simulink model "SoftGripperPick"  (R2026b)
settings: Solver=daessc  StopTime=16  RelTol=1e-4
undefined symbols (not defined in the file): magnitude, P, X, Y, Z
libraries: sm_lib x123, nesl_utility x40, fl_lib x4
(part 3 of 3)

== system SoftGripperPick/Plant/UR5e/wrist_2_link ==
  Inertia : sm_lib/Body Elements/Inertia  InertiaType=Custom  Mass=1.3  MassUnits=kg  CenterOfMass=[0, 0, 0]  CenterOfMassUnits=m  MomentsOfInertia=[0.00135617, 0.00096614, 0.00127827]  MomentsOfInertiaUnits=kg*m^2  ProductsOfInertia=[5.048000000000011e-05, 2.739999999999998e-06, 4.440000000000001e-06]  ProductsOfInertiaUnits=kg*m^2  GraphicType=None  MarkerShape=Inertia  MarkerSize=20  GraphicVisPropType=SimpleVisualProperties  GraphicDiffuseColor=[0.5 0.5 0.5]  GraphicOpacity=1  GraphicSpecularColor=[0.5 0.5 0.5 1.0]  GraphicAmbientColor=[0.15 0.15 0.15 1.0]  GraphicEmissiveColor=[0.0 0.0 0.0 1.0]  GraphicShininess=75
  InertiaOriginTransform : sm_lib/Frames and Transforms/Rigid Transform  RotationMethod=RotationSequence  FollAlignAxisA=+X  BaseAlignAxisA=+Y  FollAlignAxisB=+Y  BaseAlignAxisB=+Z  RotationStandardAxis=+Z  RotationAngle=0  RotationAngleUnits=deg  RotationArbitraryAxis=[0 0 1]  RotationSequenceAxes=BaseAxes  RotationSequence=XYZ  RotationSequenceAngles=[0, 0, 0]  RotationSequenceAnglesUnits=rad  RotationMatrix=[1 0 0;0 1 0;0 0 1]  Quaternion=[1 0 0 0]  TranslationMethod=Cartesian  TranslationCartesianOffset=[0, 0.01634, -0.0018]  TranslationCartesianOffsetUnits=m  TranslationStandardAxis=+Z  TranslationStandardOffset=0  TranslationStandardOffsetUnits=m  TranslationROffset=0  TranslationROffsetUnits=m  TranslationThetaOffset=0  TranslationThetaOffsetUnits=deg  TranslationZOffset=0  TranslationZOffsetUnits=m
  ReferenceFrame : sm_lib/Frames and Transforms/Reference Frame
  wrist_2_joint_AxisInvTransform : sm_lib/Frames and Transforms/Rigid Transform  RotationMethod=ArbitraryAxis  FollAlignAxisA=+X  BaseAlignAxisA=+Y  FollAlignAxisB=+Y  BaseAlignAxisB=+Z  RotationStandardAxis=+Z  RotationAngle=0  RotationAngleUnits=rad  RotationArbitraryAxis=[1, 0, 0]  RotationSequenceAxes=FollowerAxes  RotationSequence=XYX  RotationSequenceAngles=[0 0 0]  RotationSequenceAnglesUnits=deg  RotationMatrix=[1 0 0;0 1 0;0 0 1]  Quaternion=[1 0 0 0]  TranslationMethod=Cartesian  TranslationCartesianOffset=[0, 0, 0]  TranslationCartesianOffsetUnits=m  TranslationStandardAxis=+Z  TranslationStandardOffset=0  TranslationStandardOffsetUnits=m  TranslationROffset=0  TranslationROffsetUnits=m  TranslationThetaOffset=0  TranslationThetaOffsetUnits=deg  TranslationZOffset=0  TranslationZOffsetUnits=m
  wrist_3_joint_AxisTransform : sm_lib/Frames and Transforms/Rigid Transform  RotationMethod=ArbitraryAxis  FollAlignAxisA=+X  BaseAlignAxisA=+Y  FollAlignAxisB=+Y  BaseAlignAxisB=+Z  RotationStandardAxis=+Z  RotationAngle=0  RotationAngleUnits=rad  RotationArbitraryAxis=[1, 0, 0]  RotationSequenceAxes=FollowerAxes  RotationSequence=XYX  RotationSequenceAngles=[0 0 0]  RotationSequenceAnglesUnits=deg  RotationMatrix=[1 0 0;0 1 0;0 0 1]  Quaternion=[1 0 0 0]  TranslationMethod=Cartesian  TranslationCartesianOffset=[0, 0, 0]  TranslationCartesianOffsetUnits=m  TranslationStandardAxis=+Z  TranslationStandardOffset=0  TranslationStandardOffsetUnits=m  TranslationROffset=0  TranslationROffsetUnits=m  TranslationThetaOffset=0  TranslationThetaOffsetUnits=deg  TranslationZOffset=0  TranslationZOffsetUnits=m
  wrist_3_joint_OriginTransform : sm_lib/Frames and Transforms/Rigid Transform  RotationMethod=RotationSequence  FollAlignAxisA=+X  BaseAlignAxisA=+Y  FollAlignAxisB=+Y  BaseAlignAxisB=+Z  RotationStandardAxis=+Z  RotationAngle=0  RotationAngleUnits=deg  RotationArbitraryAxis=[0 0 1]  RotationSequenceAxes=BaseAxes  RotationSequence=XYZ  RotationSequenceAngles=[-1.570796327, 1.224646799147353e-16, -1.224646799147353e-16]  RotationSequenceAnglesUnits=rad  RotationMatrix=[1 0 0;0 1 0;0 0 1]  Quaternion=[1 0 0 0]  TranslationMethod=Cartesian  TranslationCartesianOffset=[0, 0.09959999999999999, -2.042830148012698e-11]  TranslationCartesianOffsetUnits=m  TranslationStandardAxis=+Z  TranslationStandardOffset=0  TranslationStandardOffsetUnits=m  TranslationROffset=0  TranslationROffsetUnits=m  TranslationThetaOffset=0  TranslationThetaOffsetUnits=deg  TranslationZOffset=0  TranslationZOffsetUnits=m
  F : PMIOPort  Side=Left
  F1 : PMIOPort  Port=2  Side=Right
  connections:
  wrist_3_joint_AxisTransform/LConn1 -- wrist_3_joint_OriginTransform/RConn1
  wrist_3_joint_AxisTransform/RConn1 -- F1/RConn1
  wrist_2_joint_AxisInvTransform/RConn1 -- F/RConn1
  wrist_3_joint_OriginTransform/LConn1 -- wrist_2_joint_AxisInvTransform/LConn1 -- ReferenceFrame/RConn1 -- InertiaOriginTransform/LConn1
  Inertia/RConn1 -- InertiaOriginTransform/RConn1

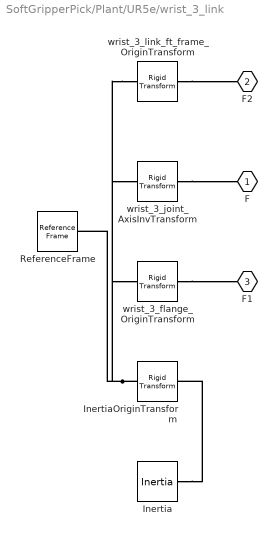
== system SoftGripperPick/Plant/UR5e/wrist_3_link ==
  Inertia : sm_lib/Body Elements/Inertia  InertiaType=Custom  Mass=0.365  MassUnits=kg  CenterOfMass=[0, 0, 0]  CenterOfMassUnits=m  MomentsOfInertia=[0.00018694, 0.00018908, 0.00025756]  MomentsOfInertiaUnits=kg*m^2  ProductsOfInertia=[-9.2e-07, -1.7e-07, 5.999999999999999e-08]  ProductsOfInertiaUnits=kg*m^2  GraphicType=None  MarkerShape=Inertia  MarkerSize=20  GraphicVisPropType=SimpleVisualProperties  GraphicDiffuseColor=[0.5 0.5 0.5]  GraphicOpacity=1  GraphicSpecularColor=[0.5 0.5 0.5 1.0]  GraphicAmbientColor=[0.15 0.15 0.15 1.0]  GraphicEmissiveColor=[0.0 0.0 0.0 1.0]  GraphicShininess=75
  InertiaOriginTransform : sm_lib/Frames and Transforms/Rigid Transform  RotationMethod=RotationSequence  FollAlignAxisA=+X  BaseAlignAxisA=+Y  FollAlignAxisB=+Y  BaseAlignAxisB=+Z  RotationStandardAxis=+Z  RotationAngle=0  RotationAngleUnits=deg  RotationArbitraryAxis=[0 0 1]  RotationSequenceAxes=BaseAxes  RotationSequence=XYZ  RotationSequenceAngles=[0, 0, 0]  RotationSequenceAnglesUnits=rad  RotationMatrix=[1 0 0;0 1 0;0 0 1]  Quaternion=[1 0 0 0]  TranslationMethod=Cartesian  TranslationCartesianOffset=[0, 0, -0.001159]  TranslationCartesianOffsetUnits=m  TranslationStandardAxis=+Z  TranslationStandardOffset=0  TranslationStandardOffsetUnits=m  TranslationROffset=0  TranslationROffsetUnits=m  TranslationThetaOffset=0  TranslationThetaOffsetUnits=deg  TranslationZOffset=0  TranslationZOffsetUnits=m
  ReferenceFrame : sm_lib/Frames and Transforms/Reference Frame
  wrist_3_flange_OriginTransform : sm_lib/Frames and Transforms/Rigid Transform  RotationMethod=RotationSequence  FollAlignAxisA=+X  BaseAlignAxisA=+Y  FollAlignAxisB=+Y  BaseAlignAxisB=+Z  RotationStandardAxis=+Z  RotationAngle=0  RotationAngleUnits=deg  RotationArbitraryAxis=[0 0 1]  RotationSequenceAxes=BaseAxes  RotationSequence=XYZ  RotationSequenceAngles=[-1.570796326794897, -1.570796326794897, 0]  RotationSequenceAnglesUnits=rad  RotationMatrix=[1 0 0;0 1 0;0 0 1]  Quaternion=[1 0 0 0]  TranslationMethod=Cartesian  TranslationCartesianOffset=[0, 0, 0]  TranslationCartesianOffsetUnits=m  TranslationStandardAxis=+Z  TranslationStandardOffset=0  TranslationStandardOffsetUnits=m  TranslationROffset=0  TranslationROffsetUnits=m  TranslationThetaOffset=0  TranslationThetaOffsetUnits=deg  TranslationZOffset=0  TranslationZOffsetUnits=m
  wrist_3_joint_AxisInvTransform : sm_lib/Frames and Transforms/Rigid Transform  RotationMethod=ArbitraryAxis  FollAlignAxisA=+X  BaseAlignAxisA=+Y  FollAlignAxisB=+Y  BaseAlignAxisB=+Z  RotationStandardAxis=+Z  RotationAngle=0  RotationAngleUnits=rad  RotationArbitraryAxis=[1, 0, 0]  RotationSequenceAxes=FollowerAxes  RotationSequence=XYX  RotationSequenceAngles=[0 0 0]  RotationSequenceAnglesUnits=deg  RotationMatrix=[1 0 0;0 1 0;0 0 1]  Quaternion=[1 0 0 0]  TranslationMethod=Cartesian  TranslationCartesianOffset=[0, 0, 0]  TranslationCartesianOffsetUnits=m  TranslationStandardAxis=+Z  TranslationStandardOffset=0  TranslationStandardOffsetUnits=m  TranslationROffset=0  TranslationROffsetUnits=m  TranslationThetaOffset=0  TranslationThetaOffsetUnits=deg  TranslationZOffset=0  TranslationZOffsetUnits=m
  wrist_3_link_ft_frame_OriginTransform : sm_lib/Frames and Transforms/Rigid Transform  RotationMethod=RotationSequence  FollAlignAxisA=+X  BaseAlignAxisA=+Y  FollAlignAxisB=+Y  BaseAlignAxisB=+Z  RotationStandardAxis=+Z  RotationAngle=0  RotationAngleUnits=deg  RotationArbitraryAxis=[0 0 1]  RotationSequenceAxes=BaseAxes  RotationSequence=XYZ  RotationSequenceAngles=[3.141592653589793, -0, 0]  RotationSequenceAnglesUnits=rad  RotationMatrix=[1 0 0;0 1 0;0 0 1]  Quaternion=[1 0 0 0]  TranslationMethod=Cartesian  TranslationCartesianOffset=[0, 0, 0]  TranslationCartesianOffsetUnits=m  TranslationStandardAxis=+Z  TranslationStandardOffset=0  TranslationStandardOffsetUnits=m  TranslationROffset=0  TranslationROffsetUnits=m  TranslationThetaOffset=0  TranslationThetaOffsetUnits=deg  TranslationZOffset=0  TranslationZOffsetUnits=m
  F : PMIOPort  Side=Left
  F2 : PMIOPort  Port=2  Side=Right
  F1 : PMIOPort  Port=3  Side=Right
  connections:
  wrist_3_link_ft_frame_OriginTransform/RConn1 -- F2/RConn1
  wrist_3_joint_AxisInvTransform/RConn1 -- F/RConn1
  wrist_3_flange_OriginTransform/RConn1 -- F1/RConn1
  wrist_3_link_ft_frame_OriginTransform/LConn1 -- wrist_3_joint_AxisInvTransform/LConn1 -- wrist_3_flange_OriginTransform/LConn1 -- ReferenceFrame/RConn1 -- InertiaOriginTransform/LConn1
  Inertia/RConn1 -- InertiaOriginTransform/RConn1

== stateflow chart SoftGripperPick/Controller/PickTask ==
  settings: updateMethod=DISCRETE  sampleTime=P.ctrl.Ts_Ctrl
  state Active
    en: Ts = taskCfg(1); pGrip = gripCfg(1); tMax = taskCfg(5);
    tTot = 0; attempt = 1; supplyLow = 0; lowCnt = 0; pCmd = 0; qCmd = qHome;
    du: tTot = tTot + Ts;
    if pCmd >= pGrip && pMeas < pGrip - gripCfg(6), lowCnt = lowCnt + 1; else, lowCnt = 0; end
    if lowCnt * Ts >= gripCfg(7), supplyLow = 1; end
    state Settle
      en: qCmd = qHome; pCmd = 0;
    state Approach
      en: tSeg = 0;
      du: tSeg = tSeg + Ts; qCmd = traj(segQ0(1,:), segQ1(1,:), segT(1), tSeg);
    state Descend
      en: tSeg = 0;
      du: tSeg = tSeg + Ts; qCmd = traj(segQ0(2,:), segQ1(2,:), segT(2), tSeg);
    state Close
      en: tC = 0; stallCnt = 0; stalled = 0; bendPrev = bend;
      du: tC = tC + Ts; pCmd = min(pGrip, pGrip * tC / gripCfg(3)); stallCnt = stallCnt + 1;
      if stallCnt >= detCfg(3), stalled = double(all(abs(bend - bendPrev) / (stallCnt * Ts) < detCfg(2))); bendPrev = bend; stallCnt = 0; end
    state CheckGrasp
      en: nContact = countContact(bend, pMeas, bendTab, detCfg);
    state Lift
      en: tSeg = 0;
      du: tSeg = tSeg + Ts; qCmd = traj(segQ0(3,:), segQ1(3,:), segT(3), tSeg);
    state Transport
      en: tSeg = 0;
      du: tSeg = tSeg + Ts; qCmd = traj(segQ0(4,:), segQ1(4,:), segT(4), tSeg);
    state Lower
      en: tSeg = 0;
      du: tSeg = tSeg + Ts; qCmd = traj(segQ0(5,:), segQ1(5,:), segT(5), tSeg);
    state Retry
      en: attempt = attempt + 1; pCmd = 0; tSeg = 0; qStart = qMeas;
      du: tSeg = tSeg + Ts; qCmd = traj(qStart, segQ0(2,:), max(segT), tSeg);
    state Release
      en: pCmd = 0;
    state Retreat
      en: tSeg = 0;
      du: tSeg = tSeg + Ts; qCmd = traj(segQ0(6,:), segQ1(6,:), segT(6), tSeg);
    (default) -> Settle
    Settle -> Approach : [after(taskCfg(2), sec)]
    Approach -> Descend : [tSeg >= segT(1) && arrived(qMeas, segQ1(1,:), taskCfg(3))]
    Descend -> Close : [tSeg >= segT(2) && arrived(qMeas, segQ1(2,:), taskCfg(3))]
    Retry -> Descend [order 2] : [tSeg >= max(segT) && arrived(qMeas, segQ0(2,:), taskCfg(3))]
    Close -> CheckGrasp [order 1] : [stalled > 0 && pMeas >= pGrip - gripCfg(2)]
    Close -> Retry [order 2] : [tC >= gripCfg(4)]
    CheckGrasp -> Lift [order 1] : [nContact >= 3]
    CheckGrasp -> Retry [order 2] : [nContact < 3]
    Lift -> Transport [order 2] : [tSeg >= segT(3) && arrived(qMeas, segQ1(3,:), taskCfg(3))]
    Lift -> Retry [order 1] : [countFree(bend, pMeas, bendTab, detCfg) >= 2]
    Transport -> Lower [order 2] : [tSeg >= segT(4) && arrived(qMeas, segQ1(4,:), taskCfg(3))]
    Transport -> Retry [order 1] : [countFree(bend, pMeas, bendTab, detCfg) >= 2]
    Lower -> Release [order 2] : [tSeg >= segT(5) && arrived(qMeas, segQ1(5,:), taskCfg(3))]
    Lower -> Retry [order 1] : [countFree(bend, pMeas, bendTab, detCfg) >= 2]
    Release -> Retreat : [after(gripCfg(5), sec)]
  state Done
    en: pCmd = 0;
    du: qCmd = qHome;
  state Failed
    en: pCmd = 0; tSeg = 0; qStart = qMeas;
    du: tSeg = tSeg + Ts; qCmd = traj(qStart, qHome, max(segT), tSeg);
  (default) -> Active
  Retry -> Failed [order 1] : [attempt > taskCfg(4)]
  Retreat -> Done : [tSeg >= segT(6) && arrived(qMeas, segQ1(6,:), taskCfg(3))]
  Active -> Failed : [tTot >= tMax]
  data: b function_input; p function_input; tab function_input; cfg function_input; n function_output; qm function_input; qt function_input; tol function_input; y function_output; q0 function_input; q1 function_input; T function_input; t function_input; q function_output; b function_input; p function_input; tab function_input; cfg function_input; n function_output; qMeas input; pMeas input; bend input; segQ0 input; segQ1 input; segT input; qHome input; gripCfg input; detCfg input; taskCfg input; bendTab input; qCmd output; pCmd output; tSeg local; tC local; tTot local; attempt local; stallCnt local; lowCnt local; supplyLow local; nContact local; bendPrev local; qStart local; Ts local; pGrip local; tMax local; stalled local
  function n = countFree(b, p, tab, cfg):
    | function n = countFree(b, p, tab, cfg)
    | % Fingers back near their free bend (the object has left them) or reading out of range: the drop detector.
    | bf = interp1(tab(1,:), tab(2,:), min(max(p, tab(1,1)), tab(1,end)));
    | valid = b >= cfg(4) & b <= cfg(5);
    | n = sum(~valid | b > bf - cfg(1));
    | end
  function y = arrived(qm, qt, tol):
    | function y = arrived(qm, qt, tol)
    | % The arm has reached the target when every joint is within tol (docs/rationale.md).
    | y = max(abs(qm(:) - qt(:))) < tol;
    | end
  function q = traj(q0, q1, T, t):
    | function q = traj(q0, q1, T, t)
    | % Minimum-jerk (quintic) interpolation q0 -> q1 over T; t is the time since the segment started.
    | s = min(max(t / T, 0), 1);
    | sig = 10*s^3 - 15*s^4 + 6*s^5;
    | q = q0(:) + (q1(:) - q0(:)) * sig;
    | end
  function n = countContact(b, p, tab, cfg):
    | function n = countContact(b, p, tab, cfg)
    | % Fingers that stopped at least dBend short of their free bend at pressure p (docs/rationale.md).
    | % cfg = [dBendContact stallRate nStall bendLo bendHi]
    | bf = interp1(tab(1,:), tab(2,:), min(max(p, tab(1,1)), tab(1,end)));
    | valid = b >= cfg(4) & b <= cfg(5);
    | n = sum(valid & b < bf - cfg(1));
    | end
